simulink model "Lab2_VM_Task_1b"  (R2024b)
settings: Solver=FixedStepDiscrete  StartTime=0.0  StopTime=Inf  FixedStep=0.02  RelTol=1e-3  EnableMultiTasking=on
undefined symbols (not defined in the file or in its folder): Angular, Linear
libraries: robotlib x3
settings Model: Creator=The MathWorks, Inc.  LastModifiedBy=david
settings SolverCC: AlgebraicLoopSolver=TrustRegion
settings DataIOCC: LimitDataPoints=on  SaveFormat=Array  ReturnWorkspaceOutputs=off
settings OptimizationCC: ZeroExternalMemoryAtStartup=off  ZeroInternalMemoryAtStartup=off  LifeSpan=Inf  MaxStackSize=64
settings DebuggingCC: SolverPrmCheckMsg=warning  UnconnectedInputMsg=warning  UnconnectedOutputMsg=warning  UnconnectedLineMsg=warning  AllowSymbolicDim=off  SFUnexpectedBacktrackingDiag=warning  SFNoUnconditionalDefaultTransitionDiag=warning  SFExecutionAtInitializationDiag=none  ArithmeticOperatorsInVariantConditions=warning
settings HardwareCC: ProdBitPerPointer=32  ProdBitPerSizeT=32  ProdBitPerPtrDiffT=32  ProdLargestAtomicFloat=None  ProdIntDivRoundTo=Undefined  ProdEndianess=Unspecified  ProdWordSize=32  ProdHWDeviceType=Generic->Unspecified (assume 32-bit Generic)  TargetHWDeviceType=Generic->Unspecified (assume 32-bit Generic)  UseEmbeddedCoderFeatures=off
settings ModelReferenceCC: EnableRefExpFcnMdlSchedulingChecks=on  PropagateSignalLabelsOutOfModel=off
settings SFSimCC: SimUseLocalCustomCode=off  CustomCodeUndefinedFunction=UseInterfaceOnly  SimTargetLang=C++
settings RTWCC: Description=Embedded Coder  SystemTargetFile=ert.tlc  HardwareBoard=Robot Operating System (ROS)  TemplateMakefile=ert_default_tmf  RTWUseLocalCustomCode=off  Toolchain=Catkin  TargetLang=C++  GPUComputeCapability=3.5
settings CodeAppCC: StateflowObjectComments=on
settings ERTTargetCC: MultiwordLength=2048  ERTCustomFileBanners=off  CodeInterfacePackaging=C++ class  SupportContinuousTime=on  SupportNonInlinedSFcns=on  RemoveResetFunc=off  SupportVariableSizeSignals=on  ModelStepFunctionPrototypeControlCompliant=off  InlinedParameterPlacement=Hierarchical  RootIOFormat=Structure reference  ConvertIfToSwitch=off  SuppressUnreachableDefaultCases=off  DynamicArrayContainerType=coder::array
settings ConfigComp: CovMetricSettings=dw  CovSaveCumulativeToWorkspaceVar=on  CovSaveSingleToWorkspaceVar=on  CovExternalEMLEnable=off  CovSFcnEnable=off

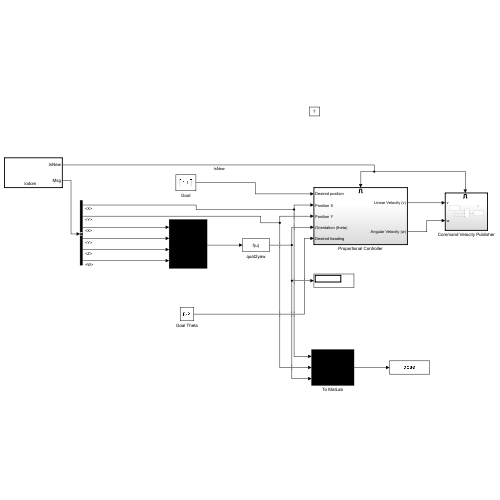
[thumbnail: Simulink's stored preview of the top-level diagram]
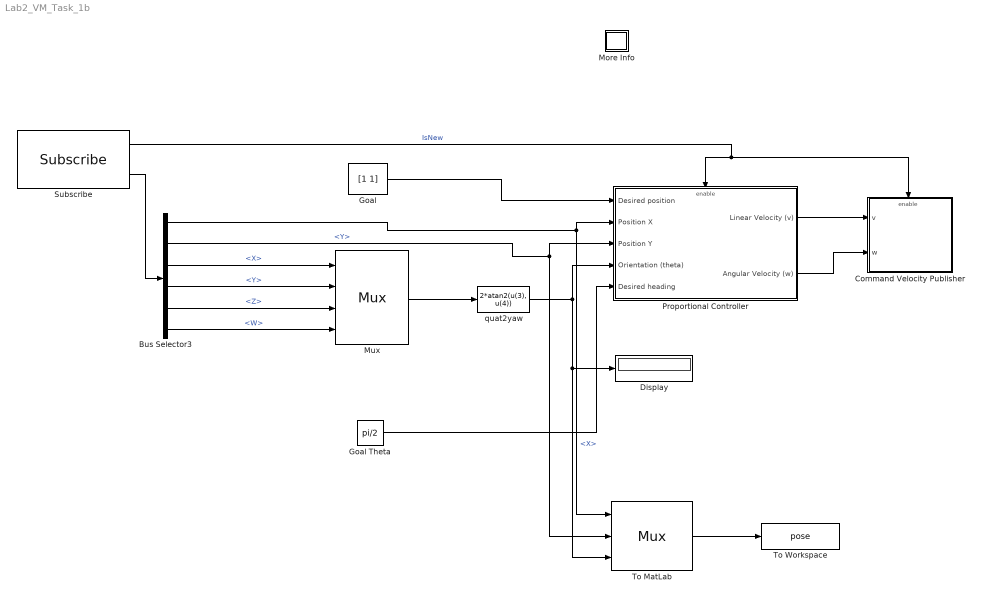
== system Lab2_VM_Task_1b ==
  Bus Selector3 : BusSelector  OutputSignals=Pose.Pose.Position.X,Pose.Pose.Position.Y,Pose.Pose.Orientation.X,Pose.Pose.Orientation.Y,Pose.Pose.Orientation.Z,Pose.Pose.Orientation.W
  Command Velocity Publisher : Subsystem
  Display : Display
  Goal : Constant  Value=[1 1]
  Goal Theta : Constant  Value=pi/2
  More Info : Subsystem
      settings: OpenFcn=showdemo(bdroot(gcb))
      mask Display: disp('?')
  Mux : Mux
  Proportional Controller : Subsystem
  Subscribe : robotlib/Subscribe  topicSource=Select from ROS network  topic=/odom  messageType=nav_msgs/Odometry  SampleTime=-1  legacyBusStruct=off  messageQueueLength=51
  To MatLab : Mux  Inputs=3
  To Workspace : ToWorkspace  VariableName=pose  SaveFormat=Timeseries  SampleTime=-1
  quat2yaw : Fcn  Expr=2*atan2(u(3), u(4))
  wires:
  Subscribe/2 -> Bus Selector3/1
  Proportional Controller/1(Linear Velocity (v)) -> Command Velocity Publisher/1(v)
  Subscribe/1 -> Command Velocity Publisher/Enable, Proportional Controller/Enable  "IsNew"
  Bus Selector3/5 -> Mux/3  "<Z>"
  Bus Selector3/6 -> Mux/4  "<W>"
  Proportional Controller/2(Angular Velocity (w)) -> Command Velocity Publisher/2(w)
  Bus Selector3/3 -> Mux/1  "<X>"
  Bus Selector3/4 -> Mux/2  "<Y>"
  Mux/1 -> quat2yaw/1
  quat2yaw/1 -> Display/1, To MatLab/3, Proportional Controller/4(Orientation (theta))
  Bus Selector3/1 -> To MatLab/1, Proportional Controller/2(Position X)  "<X>"
  Bus Selector3/2 -> To MatLab/2, Proportional Controller/3(Position Y)  "<Y>"
  Goal/1 -> Proportional Controller/1(Desired position)
  To MatLab/1 -> To Workspace/1
  Goal Theta/1 -> Proportional Controller/5(Desired heading)

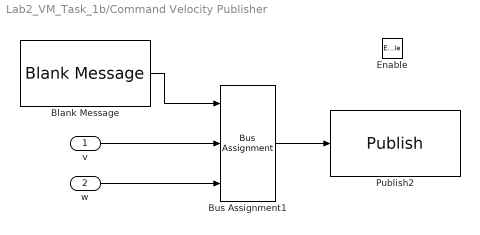
== system Lab2_VM_Task_1b/Command Velocity Publisher ==
  v : Inport
  w : Inport  Port=2
  Enable : EnablePort
  Blank Message : robotlib/Blank Message  messageClass=Message  entityType=geometry_msgs/Twist  messageType=geometry_msgs/Twist  SampleTime=inf  legacyBusStruct=off
  Bus Assignment1 : BusAssignment  DialogController=Simulink.DDGSource_BusAssignment  AssignedSignals=Linear.X,Angular.Z
  Publish2 : robotlib/Publish  topicSource=Select from ROS network  topic=/cmd_vel  messageType=geometry_msgs/Twist  legacyBusStruct=off  messageQueueLength=105
  wires:
  Bus Assignment1/1 -> Publish2/1
  Blank Message/1 -> Bus Assignment1/1
  v/1 -> Bus Assignment1/2
  w/1 -> Bus Assignment1/3

== system Lab2_VM_Task_1b/More Info ==

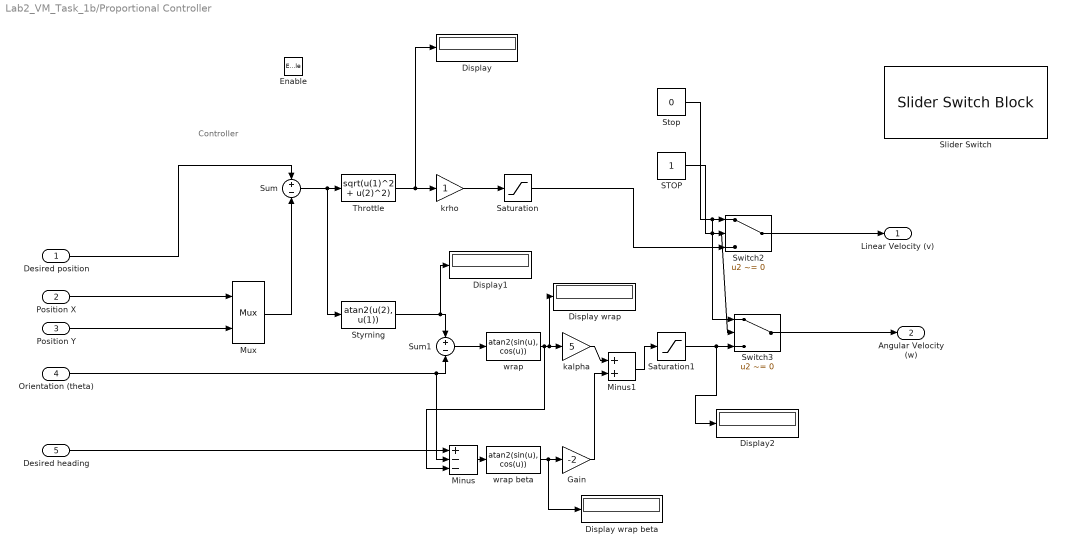
== system Lab2_VM_Task_1b/Proportional Controller ==
  note: Controller
  Desired position : Inport
  Position X : Inport  Port=2
  Position Y : Inport  Port=3
  Orientation (theta) : Inport  Port=4
  Desired heading : Inport  Port=5
  Enable : EnablePort
  Display : Display
  Display wrap : Display
  Display wrap beta : Display
  Display1 : Display
  Display2 : Display
  Gain : Gain  Gain=-2
  Minus : Sum  Inputs=+--
  Minus1 : Sum
  Mux : Mux  Inputs=2
  "STOP " : Constant
  Saturation : Saturate  UpperLimit=0.22  LowerLimit=0
  Saturation1 : Saturate  UpperLimit=2.84  LowerLimit=-2.84
  Slider Switch : SliderSwitchBlock
      settings: Values={{'Off', 'On'}, [0 1]}
  Stop : Constant  Value=0
  Styrning : Fcn  Expr=atan2(u(2), u(1))
  Sum : Sum  Inputs=+-
  Sum1 : Sum  Inputs=+-
  Switch2 : Switch  Criteria=u2 ~= 0  SaturateOnIntegerOverflow=off  InputSameDT=off
  Switch3 : Switch  Criteria=u2 ~= 0  SaturateOnIntegerOverflow=off  InputSameDT=off
  Throttle : Fcn  Expr=sqrt(u(1)^2 + u(2)^2)
  kalpha : Gain  Gain=5
  krho : Gain
  wrap : Fcn  Expr=atan2(sin(u), cos(u))
  wrap beta : Fcn  Expr=atan2(sin(u), cos(u))
  Linear Velocity (v) : Outport  VectorParamsAs1DForOutWhenUnconnected=off
  Angular Velocity (w) : Outport  Port=2  VectorParamsAs1DForOutWhenUnconnected=off
  wires:
  Stop/1 -> Switch3/1, Switch2/1
  "STOP "/1 -> Switch3/2, Switch2/2
  Switch2/1 -> Linear Velocity (v)/1
  Switch3/1 -> Angular Velocity (w)/1
  Saturation/1 -> Switch2/3
  Desired position/1 -> Sum/1
  Sum/1 -> Styrning/1, Throttle/1
  Mux/1 -> Sum/2
  Position X/1 -> Mux/1
  Position Y/1 -> Mux/2
  Throttle/1 -> Display/1, krho/1
  krho/1 -> Saturation/1
  Orientation (theta)/1 -> Minus/2, Sum1/2
  Sum1/1 -> wrap/1
  wrap/1 -> Minus/3, Display wrap/1, kalpha/1
  Saturation1/1 -> Display2/1, Switch3/3
  Styrning/1 -> Display1/1, Sum1/1
  Desired heading/1 -> Minus/1
  Minus/1 -> wrap beta/1
  wrap beta/1 -> Display wrap beta/1, Gain/1
  kalpha/1 -> Minus1/1
  Gain/1 -> Minus1/2
  Minus1/1 -> Saturation1/1
